simulink model "heli_q8_Part4_AI_Help"  (R2026a)
settings: Solver=ode1  StopTime=100  FixedStep=0.002  EnableMultiTasking=on
PostLoadFcn:
  | qc_set_target_type(getConfigSet(bdroot, 'QUARC Default Target Configuration'));
values from neighbouring files (symbols this model uses):
  A_d = sysd.A    [init_heli_3_10_Part4.m]    (also in init_heli_3_10_Part4_Improved.m = sysb.A; init_heli_3_10_Part4_Working.m)
  B_d = sysd.B    [init_heli_3_10_Part4.m]    (also in init_heli_3_10_Part4_Improved.m = sysb.B; init_heli_3_10_Part4_Working.m)
  C_d = sysd.C    [init_heli_3_10_Part4.m]    (also in init_heli_3_10_Part4_Improved.m = sysb.C; init_heli_3_10_Part4_Working.m)
  F = [K(1,1) K(1,3) ... (first row only)    [init_heli_3_10_Part4.m]    (also in init_heli_3_10_Part4_Improved.m; init_heli_3_10_Part4_Working.m)
  Joystick_gain_x = 1    [init_heli_3_10_Part4.m]    (also in init_heli_3_10_Part4_Improved.m; init_heli_3_10_Part4_Working.m)
  Joystick_gain_y = -1    [init_heli_3_10_Part4.m]    (also in init_heli_3_10_Part4_Improved.m; init_heli_3_10_Part4_Working.m)
  K = lqr(A_lqr,B_lqr,Q_lqr,R_lqr)    [init_heli_3_10_Part4.m]    (also in init_heli_3_10_Part4_Improved.m; init_heli_3_10_Part4_Working.m)
  K_pd = lambda_1*lambda_2/K_1    (= 7.56880733945)    [init_heli_3_10_Part4.m]    (also in init_heli_3_10_Part4_Improved.m; init_heli_3_10_Part4_Working.m)
  K_pp = - (lambda_1 + lambda_2)/K_1    (= 7.56880733945)    [init_heli_3_10_Part4.m]    (also in init_heli_3_10_Part4_Improved.m; init_heli_3_10_Part4_Working.m)
  P_0 = zeros(12)    [init_heli_3_10_Part4.m]    (also in init_heli_3_10_Part4_Improved.m = zeros(9); init_heli_3_10_Part4_Working.m)
  Q_d = Ad * Mx(1:n, n+1:end)    [init_heli_3_10_Part4.m]    (also in init_heli_3_10_Part4_Improved.m = blkdiag(Q_d6, diag([3e-12 6e-9 3e-12])); init_heli_3_10_Part4_Working.m)
  R_d2 = [R_d2 zeros(6) ... (first row only)    [init_heli_3_10_Part4.m]    (also in init_heli_3_10_Part4_Improved.m = diag(diag(R_full)); init_heli_3_10_Part4_Working.m = blkdiag(R_d2, 10^-3*R_d2))
  V_s0 = 7.5    [init_heli_3_10_Part4.m]    (also in init_heli_3_10_Part4_Improved.m; init_heli_3_10_Part4_Working.m)
  x_0 = [0;0;0;0;0;0 ... (first row only)    [init_heli_3_10_Part4.m]    (also in init_heli_3_10_Part4_Improved.m = [0; init_heli_3_10_Part4_Working.m)
undefined symbols (not defined in the file or in its folder): HIL, qc_get_step_size
libraries: quarc_library x9
settings Model: SimulationMode=external  ExtModeTrigDuration=5000  Creator=Rchan  LastModifiedBy=sandranb
settings SolverCC: PositivePriorityOrder=on
settings DataIOCC: SignalLoggingSaveFormat=ModelDataLogs
settings OptimizationCC: InitFltsAndDblsToZero=on
settings DebuggingCC: SaveWithParameterizedLinksMsg=none  UnderspecifiedInitializationDetection=Classic  MultiTaskDSMMsg=warning  MultiTaskCondExecSysMsg=none
settings HardwareCC: ProdHWDeviceType=32-bit Generic
settings RTWCC: SystemTargetFile=quarc_win64.tlc  TemplateMakefile=quarc_default_tmf  Description=QUARC Win64 Target
settings STFCustomTargetCC: SystemTargetFile=quarc_win64.tlc  TargetPreCompLibLocation=C:\PROGRA~3\QUARC\lib\2020b\win64\release  MultiwordLength=2048.0  ConcurrentExecutionCompliant=on  CPPClassGenCompliant=on  Debug=off  StopOnOverrun=off
settings GRTTargetCC: ExtMode=on  ExtModeMexFile=quarc_comm  TargetPreCompLibLocation=C:\PROGRA~3\QUARC\lib\2020b\win64\release  ParMdlRefBuildCompliant=off  CompOptLevelCompliant=off  CombineOutputUpdateFcns=off  MatFileLogging=off  GRTInterface=on

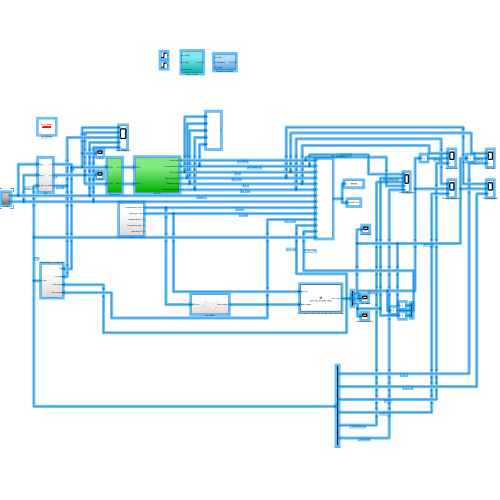
[thumbnail: Simulink's stored preview of the top-level diagram]
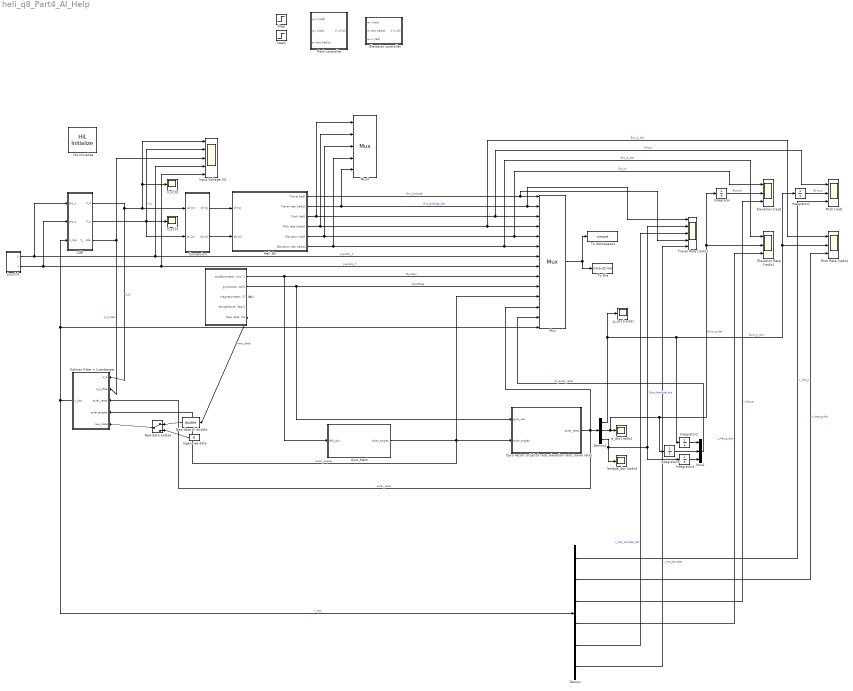
== system heli_q8_Part4_AI_Help ==
  Conversion : Subsystem
  Demux : Demux  Outputs=6
  Demux2 : Demux  Outputs=3
  Elevation Rate [rad/s] : Scope  NumInputPorts=3
      settings: ActiveDisplayYMinimum=-0.55642  ActiveDisplayYMaximum=0.56813  DataLoggingVariableName=ScopeData19
  Elevation [rad] : Scope  NumInputPorts=3
      settings: ActiveDisplayYMinimum=-0.05467  ActiveDisplayYMaximum=0.48183  DataLoggingVariableName=ScopeData18
  Elevation controller : Subsystem
  "Gyro vector to [pitch rate, elevation rate, travel rate]" : MATLAB Function  TreatAsAtomicUnit=on
  Gyro_Math : Subsystem
  HIL Initialize : quarc_library/Data Acquisition/Generic/Configuration/HIL Initialize  Priority=-99  object_name=HIL-1  board_type=q8_usb  board_number=0  board_options=update_rate=normal;decimation=1  exclusive=off  active=off  hardware_clocks=[0:2]  clock_modes=[]  initial_clock_frequencies=[]  set_clock_params_at_start=off  set_clock_params_at_switch_in=off  set_clock_frequencies_at_start=off  set_clock_frequencies_at_switch_in=off  analog_input_channels=[0:7]  analog_input_configurations=[]  analog_input_maximums=10  analog_input_minimums=-10  set_analog_input_params_at_start=on  set_analog_input_params_at_switch_in=off  analog_output_channels=[0:7]  analog_output_maximums=10  analog_output_minimums=-10  initial_analog_outputs=[0]  final_analog_outputs=[0]  watchdog_analog_outputs=0  set_analog_output_params_at_start=on  set_analog_output_params_at_switch_in=off  set_analog_outputs_at_start=on  set_analog_outputs_at_switch_in=off  set_analog_outputs_at_terminate=on  set_analog_outputs_at_switch_out=off  set_analog_outputs_on_watchdog=off  digital_input_channels=[]  digital_output_channels=[]  digital_output_configuration=[]  initial_digital_outputs=[1]  final_digital_outputs=[1]  watchdog_digital_outputs=[1]  set_digital_output_params_at_start=off  set_digital_output_params_at_switch_in=off  set_digital_outputs_at_start=on  set_digital_outputs_at_switch_in=off  set_digital_outputs_at_terminate=on  set_digital_outputs_at_switch_out=off  set_digital_outputs_on_watchdog=off  encoder_channels=[0:7]  quadrature=[4]  encoder_filter_frequency=[]  initial_encoder_counts=[0]  set_encoder_params_at_start=on  set_encoder_params_at_switch_in=off  set_encoder_counts_at_start=on  set_encoder_counts_at_switch_in=off  pwm_channels=[0:7]  pwm_modes=0  pwm_frequency=99.532799999999995e6/4095  pwm_configuration=[0]  pwm_alignment=[0]  pwm_polarity=[1]  pwm_leading_deadband=[0]  pwm_trailing_deadband=[0]  initial_pwm_outputs=[0]  final_pwm_outputs=[0]  watchdog_pwm_outputs=[0]  set_pwm_params_at_start=on  set_pwm_params_at_switch_in=off  set_pwm_outputs_at_start=on  set_pwm_outputs_at_switch_in=off  set_pwm_outputs_at_terminate=on  set_pwm_outputs_at_switch_out=off  set_pwm_outputs_on_watchdog=off  other_output_channels=[]  initial_other_outputs=[]  final_other_outputs=[]  watchdog_other_outputs=[]  set_other_outputs_at_start=off  set_other_outputs_at_switch_in=off  set_other_outputs_at_terminate=off  set_other_outputs_at_switch_out=off  set_other_outputs_on_watchdog=off
  Heli 3D : Subsystem
  IMU : Subsystem
  Input Voltage [V] : Scope  NumInputPorts=5
      settings: ActiveDisplayYMinimum=-4.40789  ActiveDisplayYMaximum=10.0852  DataLoggingVariableName=ScopeData22
  Integrator{,1..4} (5 alike) : Integrator
  Joystick : Subsystem
  Kalman Filter + Luenberger : Subsystem
  LQR : Subsystem
  Mux : Mux  Inputs=14
      settings: DisplayOption=signals
  Mux1 : Mux  Inputs=3
  Mux3 : Mux  Inputs=5
      settings: DisplayOption=signals
  Pitch Rate [rad/s] : Scope  NumInputPorts=3
      settings: ActiveDisplayYMinimum=-0.34541  ActiveDisplayYMaximum=0.52446  DataLoggingVariableName=ScopeData21
  Pitch [rad] : Scope  NumInputPorts=3
      settings: ActiveDisplayYMinimum=-0.33937  ActiveDisplayYMaximum=0.18576  DataLoggingVariableName=ScopeData20
  Pitch controller : Subsystem
  Step : Step  Time=5  FinalValue=0.5  SampleTime=0
  Step1 : Step  Time=5  FinalValue=0  SampleTime=0
  To File : ToFile  Filename=simout2.mat
  To Workspace1 : ToWorkspace  VariableName=simout  SaveFormat=Structure With Time  SampleTime=-1
  Travel Rate [rad/s] : Scope  NumInputPorts=5
      settings: ActiveDisplayYMinimum=-0.51279  ActiveDisplayYMaximum=0.73956  DataLoggingVariableName=ScopeData17
  V_d [V] : Scope
      settings: ActiveDisplayYMinimum=-0.95758  ActiveDisplayYMaximum=0.62672  DataLoggingVariableName=ScopeData13
  V_s [V] : Scope
      settings: ActiveDisplayYMinimum=-1.07949  ActiveDisplayYMaximum=9.71538  DataLoggingVariableName=ScopeData14
  e_dot [rad/s] : Scope
      settings: ActiveDisplayYMinimum=-0.55031  ActiveDisplayYMaximum=0.82946  DataLoggingVariableName=ScopeData4
  lambda_dot [rad/s] : Scope
      settings: ActiveDisplayYMinimum=-0.51279  ActiveDisplayYMaximum=0.73956  DataLoggingVariableName=ScopeData5
  p_dot [rad/s] : Scope
      settings: ActiveDisplayYMinimum=-0.32422  ActiveDisplayYMaximum=0.52211  DataLoggingVariableName=ScopeData3
  New data av/paa : ManualSwitch
  Ingen nye data : Constant  Value=0
  New data til double : DataTypeConversion  OutDataTypeStr=double  SaturateOnIntegerOverflow=off  RndMeth=Floor
  wires:
  Conversion/2(Vb [V]) -> Heli 3D/2(Vb [V])
  Conversion/1(Vf [V]) -> Heli 3D/1(Vf [V])
  Heli 3D/1(Travel [rad]) -> Travel Rate [rad/s]/4, Mux/1  "Enc_lambda"
  Heli 3D/2(Travel rate [rad/s]) -> Travel Rate [rad/s]/1, Mux/2, Mux3/5  "Enc_lambda_dot"
  Heli 3D/3(Pitch [rad]) -> Mux/3, Pitch [rad]/1, Mux3/1  "Enc_p"
  Heli 3D/4(Pitch rate [rad/s]) -> Pitch Rate [rad/s]/1, Mux/4, Mux3/2  "Enc_p_dot"
  Heli 3D/5(Elevation [rad]) -> Elevation [rad]/1, Mux/5, Mux3/3  "Enc_e"
  Heli 3D/6(Elevation rate [rad/s]) -> Elevation Rate [rad/s]/1, Mux/6, Mux3/4  "Enc_e_dot"
  Mux/1 -> To Workspace1/1, To File/1
  Joystick/1(X) -> Mux/7, Input Voltage [V]/4, LQR/1(Joy_x)  "Joystick_X"
  Joystick/2(Y) -> LQR/2(Joy_y), Mux/8, Input Voltage [V]/5  "Joystick_Y"
  IMU/1("accelerometer, m/s^2") -> Gyro_Math/1(IMU_Acc), Mux/9  "GyroAcc"
  IMU/2("gyroscope, rad/s") -> Mux/10, "Gyro vector to [pitch rate, elevation rate, travel rate]"/1(gyro_vec)  "GyroRate"
  "Gyro vector to [pitch rate, elevation rate, travel rate]"/1(euler_rates) -> Mux/12, Kalman Filter + Luenberger/3(euler_rates), Demux2/1  "euler_rates"
  Demux2/3 -> Integrator4/1, Travel Rate [rad/s]/2, lambda_dot [rad/s]/1  "Gyro_lambda_dot"
  Demux2/2 -> Integrator3/1, Elevation Rate [rad/s]/2, Integrator/1, e_dot [rad/s]/1  "Gyro_e_dot"
  Demux2/1 -> Integrator2/1, Integrator1/1, Pitch Rate [rad/s]/2, p_dot [rad/s]/1  "Gyro_p_dot"
  Gyro_Math/1(euler_angles) -> Mux/11, Kalman Filter + Luenberger/4(euler_angles), "Gyro vector to [pitch rate, elevation rate, travel rate]"/2(euler_angles)  "euler_angles"
  LQR/1(V_d) -> Conversion/1(Vd [V]), V_d [V]/1, Input Voltage [V]/1, Kalman Filter + Luenberger/1(V_d)  "V_d"
  LQR/2(V_s) -> V_s [V]/1, Conversion/2(Vs [V]), Input Voltage [V]/2  "V_s"
  Kalman Filter + Luenberger/1(x_hat) -> Mux/14, LQR/3(x_hat), Demux/1  "x_hat"
  Demux/5 -> Travel Rate [rad/s]/3  "x_hat_lambda_dot"
  Demux/3 -> Elevation [rad]/3  "x_hat_e"
  Integrator/1 -> Elevation [rad]/2  "Gyro_e"
  Demux/4 -> Elevation Rate [rad/s]/3  "x_hat_e_dot"
  Integrator1/1 -> Pitch [rad]/2  "Gyro_p"
  Demux/2 -> Pitch Rate [rad/s]/3  "x_hat_p_dot"
  Demux/1 -> Pitch [rad]/3  "x_hat_p"
  LQR/3(V_s_tilde) -> Input Voltage [V]/3, Kalman Filter + Luenberger/2(V_s_tilde)  "V_s_tilde"
  Integrator2/1 -> Mux1/1
  Integrator4/1 -> Mux1/3
  Integrator3/1 -> Mux1/2
  Mux1/1 -> Mux/13  "int_euler_rates"
  Demux/6 -> Travel Rate [rad/s]/5  "x_hat_lambda"
  IMU/5("New data, 0/1") -> New data til double/1  "new_data"
  New data til double/1 -> New data av/paa/1
  Ingen nye data/1 -> New data av/paa/2
  New data av/paa/1 -> Kalman Filter + Luenberger/5(new_data)

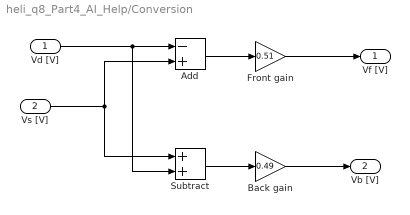
== system heli_q8_Part4_AI_Help/Conversion ==
  Vd [V] : Inport
  Vs [V] : Inport  Port=2
  Add : Sum  Inputs=-+
  Back gain : Gain  Gain=0.49
  Front gain : Gain  Gain=0.51
  Subtract : Sum
  Vf [V] : Outport
  Vb [V] : Outport  Port=2
  wires:
  Vd [V]/1 -> Subtract/2, Add/1
  Vs [V]/1 -> Subtract/1, Add/2
  Subtract/1 -> Back gain/1
  Back gain/1 -> Vb [V]/1
  Add/1 -> Front gain/1
  Front gain/1 -> Vf [V]/1

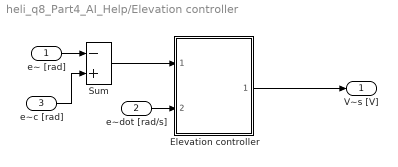
== system heli_q8_Part4_AI_Help/Elevation controller ==
  e~ [rad] : Inport
  e~dot [rad/s] : Inport  Port=2
  e~c [rad] : Inport  Port=3
  Elevation controller : Subsystem
  Sum : Sum  Inputs=-+  InputSameDT=on  SaturateOnIntegerOverflow=on  OutDataTypeStr=Inherit: Same as first input
  V~s [V] : Outport  InitialOutput=0
  wires:
  Sum/1 -> Elevation controller/1(e~ [rad])
  Elevation controller/1(V~_s [V]) -> V~s [V]/1
  e~ [rad]/1 -> Sum/1
  e~dot [rad/s]/1 -> Elevation controller/2(e~_dot [rad/s])
  e~c [rad]/1 -> Sum/2

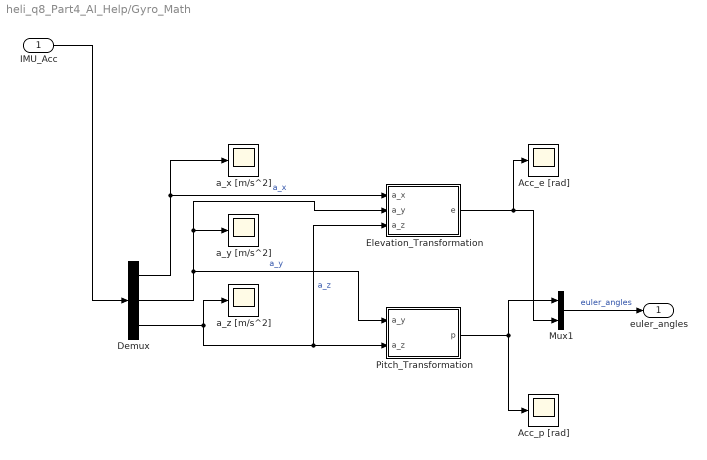
== system heli_q8_Part4_AI_Help/Gyro_Math ==
  IMU_Acc : Inport
  Acc_e [rad] : Scope
      settings: ActiveDisplayYMinimum=-0.55561  ActiveDisplayYMaximum=2.33684  DataLoggingVariableName=ScopeData2
  Acc_p [rad] : Scope
      settings: ActiveDisplayYMinimum=-0.65836  ActiveDisplayYMaximum=1.81848
  Demux : Demux  Outputs=3
  Elevation_Transformation : MATLAB Function  TreatAsAtomicUnit=on
  Mux1 : Mux  Inputs=2
  Pitch_Transformation : MATLAB Function  TreatAsAtomicUnit=on
  a_x [m/s^2] : Scope
      settings: ActiveDisplayYMinimum=-10.05504  ActiveDisplayYMaximum=6.79576
  a_y [m/s^2] : Scope
      settings: ActiveDisplayYMinimum=-2.46286  ActiveDisplayYMaximum=4.78296  DataLoggingVariableName=ScopeData2
  a_z [m/s^2] : Scope
      settings: ActiveDisplayYMinimum=-17.95765  ActiveDisplayYMaximum=1.99529  DataLoggingVariableName=ScopeData3
  euler_angles : Outport
  wires:
  Demux/1 -> a_x [m/s^2]/1, Elevation_Transformation/1(a_x)  "a_x"
  Demux/2 -> Elevation_Transformation/2(a_y), a_y [m/s^2]/1, Pitch_Transformation/1(a_y)  "a_y"
  Pitch_Transformation/1(p) -> Mux1/1, Acc_p [rad]/1
  Demux/3 -> a_z [m/s^2]/1, Elevation_Transformation/3(a_z), Pitch_Transformation/2(a_z)  "a_z"
  Elevation_Transformation/1(e) -> Acc_e [rad]/1, Mux1/2
  IMU_Acc/1 -> Demux/1
  Mux1/1 -> euler_angles/1  "euler_angles"

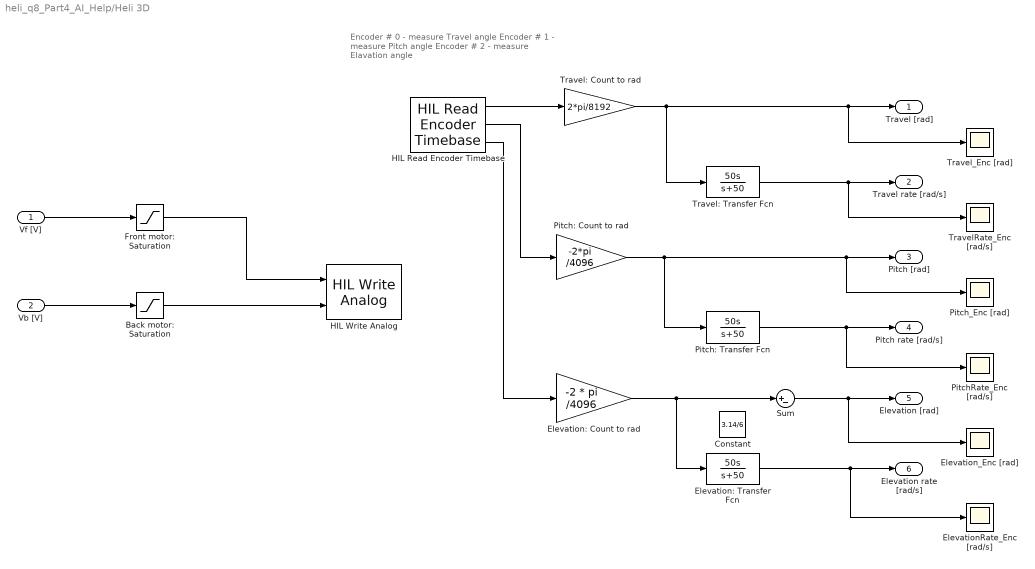
== system heli_q8_Part4_AI_Help/Heli 3D ==
  note: Encoder # 0 - measure Travel angle
      | Encoder # 1 - measure Pitch angle
      | Encoder # 2 - measure Elavation angle
  Vf [V] : Inport
  Vb [V] : Inport  Port=2
  Back motor: Saturation : Saturate  UpperLimit=5  LowerLimit=-5
  Constant : Constant  Value=3.14/6
  Elevation: Count to rad : Gain  Gain=-2 * pi /4096
  Elevation: Transfer Fcn : TransferFcn  Numerator=[50 0]  Denominator=[1 50]
  ElevationRate_Enc [rad/s] : Scope
      settings: ActiveDisplayYMinimum=-0.13148  ActiveDisplayYMaximum=0.37559  DataLoggingVariableName=ScopeData11
  Elevation_Enc [rad] : Scope
      settings: ActiveDisplayYMinimum=-0.05235  ActiveDisplayYMaximum=0.47112  DataLoggingVariableName=ScopeData10
  Front motor: Saturation : Saturate  UpperLimit=5  LowerLimit=-5
  HIL Read Encoder Timebase : quarc_library/Data Acquisition/Generic/Timebases/HIL Read Encoder Timebase  object_name=HIL-1  clock=0  channels=[0:2]  active=on  vector_output=off  data_type_mode=Inherit via back propagation  data_type=double  overflow_mode=Error on overflow  samples_in_buffer=max(ceil(1/qc_get_step_size), 1)
  HIL Write Analog : quarc_library/Data Acquisition/Generic/Immediate I//O/HIL Write Analog  object_name=HIL-1  channels=[0:1]  sample_time=-1  active=off  vector_input=off
  Pitch: Count to rad : Gain  Gain=-2*pi /4096
  Pitch: Transfer Fcn : TransferFcn  Numerator=[50 0]  Denominator=[1 50]
  PitchRate_Enc [rad/s] : Scope
      settings: ActiveDisplayYMinimum=-0.3153  ActiveDisplayYMaximum=0.25341  DataLoggingVariableName=ScopeData9
  Pitch_Enc [rad] : Scope
      settings: ActiveDisplayYMinimum=-0.33268  ActiveDisplayYMaximum=0.12559  DataLoggingVariableName=ScopeData8
  Sum : Sum  Inputs=|+-
  Travel: Count to rad : Gain  Gain=2*pi/8192
  Travel: Transfer Fcn : TransferFcn  Numerator=[50 0]  Denominator=[1 50]
  TravelRate_Enc [rad/s] : Scope
      settings: ActiveDisplayYMinimum=-0.28865  ActiveDisplayYMaximum=0.26091  DataLoggingVariableName=ScopeData7
  Travel_Enc [rad] : Scope
      settings: ActiveDisplayYMinimum=-0.31974  ActiveDisplayYMaximum=0.42328  DataLoggingVariableName=ScopeData6
  Travel [rad] : Outport
  Travel rate [rad/s] : Outport  Port=2
  Pitch [rad] : Outport  Port=3
  Pitch rate [rad/s] : Outport  Port=4
  Elevation [rad] : Outport  Port=5
  Elevation rate [rad/s] : Outport  Port=6
  wires:
  HIL Read Encoder Timebase/1 -> Travel: Count to rad/1
  HIL Read Encoder Timebase/2 -> Pitch: Count to rad/1
  HIL Read Encoder Timebase/3 -> Elevation: Count to rad/1
  Travel: Count to rad/1 -> Travel [rad]/1, Travel_Enc [rad]/1, Travel: Transfer Fcn/1
  Travel: Transfer Fcn/1 -> TravelRate_Enc [rad/s]/1, Travel rate [rad/s]/1
  Pitch: Count to rad/1 -> Pitch: Transfer Fcn/1, Pitch_Enc [rad]/1, Pitch [rad]/1
  Pitch: Transfer Fcn/1 -> PitchRate_Enc [rad/s]/1, Pitch rate [rad/s]/1
  Elevation: Count to rad/1 -> Sum/1, Elevation: Transfer Fcn/1
  Elevation: Transfer Fcn/1 -> ElevationRate_Enc [rad/s]/1, Elevation rate [rad/s]/1
  Vf [V]/1 -> Front motor: Saturation/1
  Vb [V]/1 -> Back motor: Saturation/1
  Front motor: Saturation/1 -> HIL Write Analog/1
  Back motor: Saturation/1 -> HIL Write Analog/2
  Sum/1 -> Elevation_Enc [rad]/1, Elevation [rad]/1

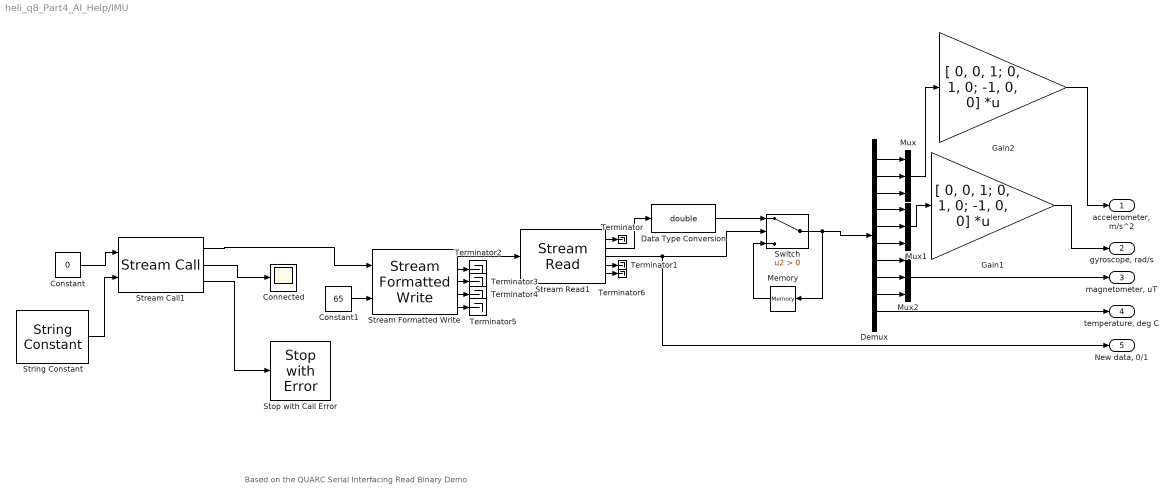
== system heli_q8_Part4_AI_Help/IMU ==
  note: Based on the QUARC Serial Interfacing Read Binary Demo
  Connected : Scope
      settings: DataLoggingVariableName=ScopeData6
  Constant : Constant  Value=0
  Constant1 : Constant  Value=65
  Data Type Conversion : DataTypeConversion  OutDataTypeStr=double  SaturateOnIntegerOverflow=off  RndMeth=Floor
  Demux : Demux  Outputs=10
  Gain1 : Gain  Gain=[ 0, 0, 1; 0, 1, 0; -1, 0, 0]  Multiplication=Matrix(K*u) (u vector)
  Gain2 : Gain  Gain=[ 0, 0, 1; 0, 1, 0; -1, 0, 0]  Multiplication=Matrix(K*u) (u vector)
  Memory : Memory  InitialCondition=[0 0 0 0 0 0 0 0 0 0]
  Mux : Mux  Inputs=3
  Mux1 : Mux  Inputs=3
  Mux2 : Mux  Inputs=3
  Stop with Call Error : quarc_library/Sinks/Error Handling/Stop with Error  message_type=Interpret input as error code  message=Error occurred
      settings: SourceProductName=QUARC Targets
  Stream Call1 : quarc_library/Communications/Intermediate/Stream Call  uri_source=External input port  uri=serial://IMU:9?baud=115200,word=8,parity=none,stop=1,flow='none'  apply_uri_to_all_configs=on  send_buffer_size=8000  receive_buffer_size=8000  byte_order=little endian (Intel - LSB first)  sample_time=qc_get_step_size  non_blocking=on  active=off
      settings: SourceProductName=QUARC Targets
  Stream Formatted Write : quarc_library/Communications/Intermediate/Stream Formatted Write  format_string=%c\n  max_code_units=80  optimization=Minimizing latency
      settings: SourceProductName=QUARC Targets
  Stream Read1 : quarc_library/Communications/Intermediate/Stream Read  data_type=single  type_expr=BusObject  num_elements=10  receive_dims=off
      settings: SourceProductName=QUARC Targets
  String Constant : quarc_library/Strings/String Constant  string_value=qc_perform_substitutions('serial://IMU:%{PORT}?baud=115200,word=8,parity=none,stop=1')  evaluate_string=on  string_type=URI  max_length=255  sample_time=inf  variable_size=off
      settings: AttributesFormatString="\"serial://IMU:6?baud=115200,word=8,parity=none,stop=1\""  SourceProductName=QUARC Targets
  Switch : Switch  Criteria=u2 > Threshold  SaturateOnIntegerOverflow=off  InputSameDT=off
  Terminator{,1..6} (7 alike) : Terminator
  "accelerometer, m/s^2" : Outport
  "gyroscope, rad/s" : Outport  Port=2
  "magnetometer, uT" : Outport  Port=3
  "temperature, deg C" : Outport  Port=4
  "New data, 0/1" : Outport  Port=5
  wires:
  Switch/1 -> Memory/1, Demux/1
  Data Type Conversion/1 -> Switch/1
  Stream Read1/3 -> "New data, 0/1"/1, Switch/2
  Stream Formatted Write/1 -> Stream Read1/1
  Constant1/1 -> Stream Formatted Write/2
  Gain1/1 -> "gyroscope, rad/s"/1
  Gain2/1 -> "accelerometer, m/s^2"/1
  Stream Read1/4 -> Terminator1/1
  Demux/10 -> "temperature, deg C"/1
  Mux1/1 -> Gain1/1
  Stream Read1/2 -> Data Type Conversion/1
  Demux/7 -> Mux2/1
  Demux/8 -> Mux2/2
  Demux/9 -> Mux2/3
  Mux2/1 -> "magnetometer, uT"/1
  Demux/6 -> Mux1/3
  Demux/5 -> Mux1/2
  Demux/4 -> Mux1/1
  Mux/1 -> Gain2/1
  Demux/3 -> Mux/3
  Demux/1 -> Mux/1
  Demux/2 -> Mux/2
  Stream Read1/1 -> Terminator/1
  Stream Call1/1 -> Stream Formatted Write/1
  Constant/1 -> Stream Call1/1
  String Constant/1 -> Stream Call1/2
  Stream Call1/2 -> Connected/1
  Stream Call1/3 -> Stop with Call Error/1
  Memory/1 -> Switch/3
  Stream Formatted Write/2 -> Terminator2/1
  Stream Formatted Write/3 -> Terminator3/1
  Stream Formatted Write/4 -> Terminator4/1
  Stream Formatted Write/5 -> Terminator5/1
  Stream Read1/5 -> Terminator6/1

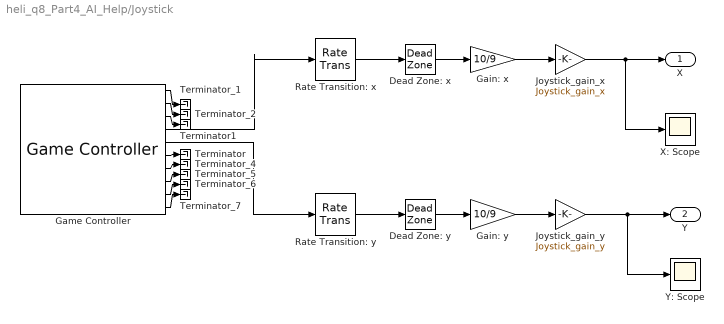
== system heli_q8_Part4_AI_Help/Joystick ==
  Dead Zone: x : DeadZone  LowerValue=-0.1  UpperValue=0.1
  Dead Zone: y : DeadZone  LowerValue=-0.1  UpperValue=0.1
  Gain: x : Gain  Gain=10/9
  Gain: y : Gain  Gain=10/9
  Game Controller : quarc_library/Devices/Peripherals/Target/Game Controller  controller=1  buffer_size=12  deadzone=[]  saturation=[]  sample_time=max(qc_get_step_size, 0.01)  auto_center=off  enabled=on
      settings: SourceProductName=QUARC Targets
  Joystick_gain_x : Gain  Gain=Joystick_gain_x
  Joystick_gain_y : Gain  Gain=Joystick_gain_y
  Rate Transition: x : RateTransition
  Rate Transition: y : RateTransition
  Terminator : Terminator
  Terminator1 : Terminator
  Terminator_{1..2,4..7} (6 alike) : Terminator
  X: Scope : Scope
      settings: ActiveDisplayYMinimum=-1  ActiveDisplayYMaximum=1  DataLoggingVariableName=ScopeData7
  Y: Scope : Scope
      settings: DataLoggingVariableName=ScopeData5
  X : Outport
  Y : Outport  Port=2
  wires:
  Rate Transition: y/1 -> Dead Zone: y/1
  Rate Transition: x/1 -> Dead Zone: x/1
  Game Controller/5 -> Rate Transition: y/1
  Game Controller/4 -> Rate Transition: x/1
  Game Controller/1 -> Terminator_1/1
  Game Controller/2 -> Terminator_2/1
  Game Controller/7 -> Terminator_4/1
  Game Controller/8 -> Terminator_5/1
  Game Controller/9 -> Terminator_6/1
  Game Controller/10 -> Terminator_7/1
  Game Controller/3 -> Terminator1/1
  Game Controller/6 -> Terminator/1
  Dead Zone: x/1 -> Gain: x/1
  Dead Zone: y/1 -> Gain: y/1
  Gain: x/1 -> Joystick_gain_x/1
  Gain: y/1 -> Joystick_gain_y/1
  Joystick_gain_x/1 -> X/1, X: Scope/1
  Joystick_gain_y/1 -> Y: Scope/1, Y/1

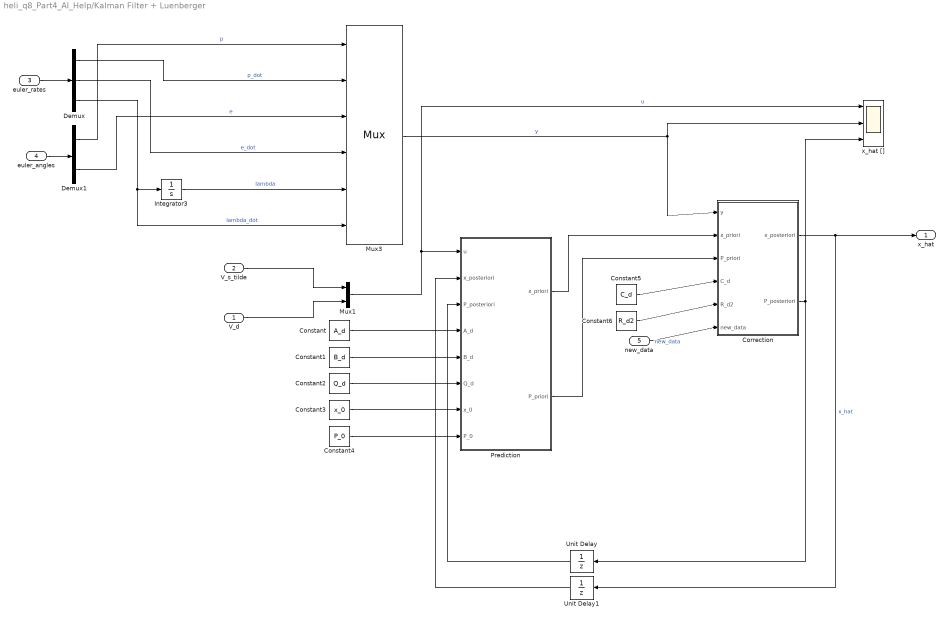
== system heli_q8_Part4_AI_Help/Kalman Filter + Luenberger ==
  V_d : Inport
  V_s_tilde : Inport  Port=2
  euler_rates : Inport  Port=3
  new_data : Inport  Port=5
  euler_angles : Inport  Port=4
  Constant : Constant  Value=A_d
  Constant1 : Constant  Value=B_d
  Constant2 : Constant  Value=Q_d
  Constant3 : Constant  Value=x_0
  Constant4 : Constant  Value=P_0
  Constant5 : Constant  Value=C_d
  Constant6 : Constant  Value=R_d2
  Correction : MATLAB Function  TreatAsAtomicUnit=on
  Demux : Demux  Outputs=3
  Demux1 : Demux  Outputs=2
  Integrator3 : Integrator
  Mux1 : Mux  Inputs=2
  Mux3 : Mux  Inputs=6
      settings: DisplayOption=signals
  Prediction : MATLAB Function  TreatAsAtomicUnit=on
  Unit Delay : UnitDelay  SampleTime=-1
  Unit Delay1 : UnitDelay  SampleTime=-1
  x_hat [] : Scope  NumInputPorts=3
      settings: ActiveDisplayYMinimum=-0.64788  ActiveDisplayYMaximum=0.72192  DataLoggingVariableName=ScopeData12
  x_hat : Outport
  wires:
  Mux3/1 -> Correction/1(y), x_hat []/2  "y"
  V_s_tilde/1 -> Mux1/1
  V_d/1 -> Mux1/2
  euler_rates/1 -> Demux/1
  Demux/1 -> Mux3/2  "p_dot"
  Demux/2 -> Mux3/4  "e_dot"
  Demux/3 -> Integrator3/1, Mux3/6  "lambda_dot"
  Integrator3/1 -> Mux3/5  "lambda"
  Mux1/1 -> x_hat []/1, Prediction/1(u)  "u"
  Prediction/1(x_priori) -> Correction/2(x_priori)
  Prediction/2(P_priori) -> Correction/3(P_priori)
  Correction/1(x_posteriori) -> Unit Delay1/1, x_hat/1  "x_hat"
  Unit Delay1/1 -> Prediction/2(x_posteriori)
  Unit Delay/1 -> Prediction/3(P_posteriori)
  Correction/2(P_posteriori) -> Unit Delay/1, x_hat []/3
  Constant/1 -> Prediction/4(A_d)
  Constant1/1 -> Prediction/5(B_d)
  Constant2/1 -> Prediction/6(Q_d)
  Constant3/1 -> Prediction/7(x_0)
  Constant4/1 -> Prediction/8(P_0)
  Constant5/1 -> Correction/4(C_d)
  Constant6/1 -> Correction/5(R_d2)
  euler_angles/1 -> Demux1/1
  Demux1/1 -> Mux3/1  "p"
  Demux1/2 -> Mux3/3  "e"
  new_data/1 -> Correction/6(new_data)  "new_data"

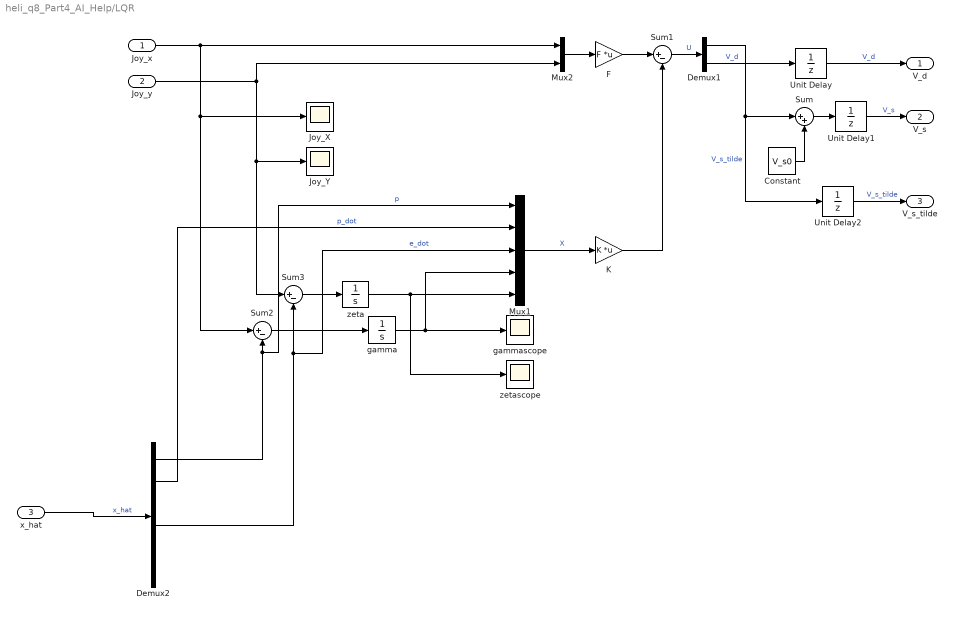
== system heli_q8_Part4_AI_Help/LQR ==
  Joy_x : Inport
  Joy_y : Inport  Port=2
  x_hat : Inport  Port=3
  Constant : Constant  Value=V_s0
  Demux1 : Demux  Outputs=2
  Demux2 : Demux  Outputs=6
  F : Gain  Gain=F  Multiplication=Matrix(K*u)
  Joy_X : Scope
      settings: ActiveDisplayYMinimum=-1  ActiveDisplayYMaximum=1
  Joy_Y : Scope
      settings: ActiveDisplayYMinimum=-1  ActiveDisplayYMaximum=1  DataLoggingVariableName=ScopeData2
  K : Gain  Gain=K  Multiplication=Matrix(K*u)
  Mux1 : Mux  Inputs=5
  Mux2 : Mux  Inputs=2
  Sum : Sum  Inputs=|++
  Sum1 : Sum  Inputs=|+-
  Sum2 : Sum  Inputs=|+-
  Sum3 : Sum  Inputs=|+-
  Unit Delay : UnitDelay  SampleTime=-1
  Unit Delay1 : UnitDelay  SampleTime=-1
  Unit Delay2 : UnitDelay  SampleTime=-1
  gamma : Integrator
  gammascope : Scope
      settings: ActiveDisplayYMinimum=-7.81453  ActiveDisplayYMaximum=1.31082  DataLoggingVariableName=ScopeData5
  zeta : Integrator
  zetascope : Scope
      settings: ActiveDisplayYMinimum=-0.42727  ActiveDisplayYMaximum=0.04825  DataLoggingVariableName=ScopeData6
  V_d : Outport
  V_s : Outport  Port=2
  V_s_tilde : Outport  Port=3
  wires:
  F/1 -> Sum1/1
  zeta/1 -> zetascope/1, Mux1/5
  gamma/1 -> Mux1/4, gammascope/1
  Sum2/1 -> gamma/1
  Mux2/1 -> F/1
  Mux1/1 -> K/1  "X"
  K/1 -> Sum1/2
  Joy_y/1 -> Mux2/2, Joy_Y/1, Sum3/1
  Sum1/1 -> Demux1/1  "U"
  Sum3/1 -> zeta/1
  Unit Delay/1 -> V_d/1  "V_d"
  Constant/1 -> Sum/2
  Demux1/1 -> Sum/1, Unit Delay2/1  "V_s_tilde"
  Sum/1 -> Unit Delay1/1
  Joy_x/1 -> Joy_X/1, Sum2/1, Mux2/1
  x_hat/1 -> Demux2/1  "x_hat"
  Demux2/4 -> Mux1/3, Sum3/2  "e_dot"
  Demux2/1 -> Mux1/1, Sum2/2  "p"
  Demux2/2 -> Mux1/2  "p_dot"
  Demux1/2 -> Unit Delay/1  "V_d"
  Unit Delay1/1 -> V_s/1  "V_s"
  Unit Delay2/1 -> V_s_tilde/1  "V_s_tilde"

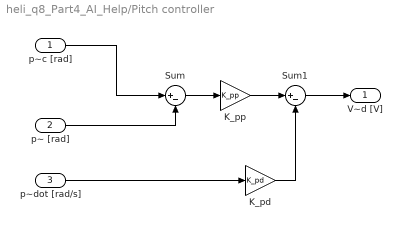
== system heli_q8_Part4_AI_Help/Pitch controller ==
  p~c [rad] : Inport
  p~ [rad] : Inport  Port=2
  p~dot [rad/s] : Inport  Port=3
  K_pd : Gain  Gain=K_pd
  K_pp : Gain  Gain=K_pp
  Sum : Sum  Inputs=|+-
  Sum1 : Sum  Inputs=|+-
  V~d [V] : Outport  InitialOutput=0
  wires:
  p~c [rad]/1 -> Sum/1
  p~ [rad]/1 -> Sum/2
  Sum/1 -> K_pp/1
  K_pp/1 -> Sum1/1
  p~dot [rad/s]/1 -> K_pd/1
  K_pd/1 -> Sum1/2
  Sum1/1 -> V~d [V]/1

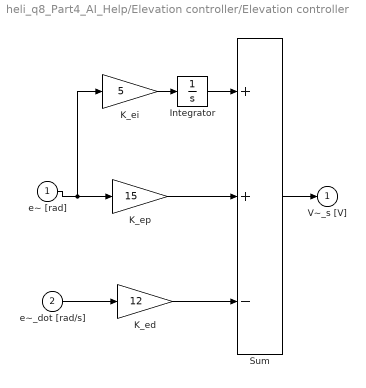
== system heli_q8_Part4_AI_Help/Elevation controller/Elevation controller ==
  e~ [rad] : Inport
  e~_dot [rad/s] : Inport  Port=2
  Integrator : Integrator  LimitOutput=on
  K_ed : Gain  Gain=12  SaturateOnIntegerOverflow=on  OutDataTypeStr=Inherit: Same as input  ParamDataTypeStr=Inherit: Same as input
  K_ei : Gain  Gain=5  SaturateOnIntegerOverflow=on  OutDataTypeStr=Inherit: Same as input  ParamDataTypeStr=Inherit: Same as input
  K_ep : Gain  Gain=15  SaturateOnIntegerOverflow=on  OutDataTypeStr=Inherit: Same as input  ParamDataTypeStr=Inherit: Same as input
  Sum : Sum  Inputs=++-  InputSameDT=on  SaturateOnIntegerOverflow=on  OutDataTypeStr=Inherit: Same as first input
  V~_s [V] : Outport  InitialOutput=0
  wires:
  K_ei/1 -> Integrator/1
  Integrator/1 -> Sum/1
  Sum/1 -> V~_s [V]/1
  e~_dot [rad/s]/1 -> K_ed/1
  K_ed/1 -> Sum/3
  K_ep/1 -> Sum/2
  e~ [rad]/1 -> K_ep/1, K_ei/1

== matlab function heli_q8_Part4_AI_Help/Gyro_Math/Elevation_Transformation ==
  data: a_x input; e output; a_y input; a_z input
function e = fcn(a_x, a_y, a_z)

N = sqrt(a_y^2+a_z^2);

if N == 0
    e = pi/2;
else
    e = atan(a_x/N);
end

== matlab function heli_q8_Part4_AI_Help/Gyro_Math/Pitch_Transformation ==
  data: a_y input; p output; a_z input
function p = fcn(a_y, a_z)

if (a_z == 0)
    p = pi/2;
else
    p = atan(a_y/a_z);
end

== matlab function heli_q8_Part4_AI_Help/Gyro vector to [pitch rate, elevation rate, travel rate] ==
  data: gyro_vec input; euler_rates output; euler_angles input
function euler_rates = gyro_vec_to_euler_rates(gyro_vec,euler_angles)
%#codegen
    phi = euler_angles(1);
    theta = euler_angles(2);
    % Hold theta unna +-pi/2 (vibrasjon ga e_acc = pi/2 og 1/cos(theta) eksploderte)
    theta = max(min(theta, 1.2), -1.2);


    T = [1, sin(phi)*tan(theta), cos(phi)*tan(theta);
         0, cos(phi),            -sin(phi);
         0, sin(phi)/cos(theta), cos(phi)/cos(theta)]; 
euler_rates = T*gyro_vec;

== matlab function heli_q8_Part4_AI_Help/Kalman Filter + Luenberger/Prediction ==
  data: u input; x_priori output; x_posteriori input; P_posteriori input; P_priori output; A_d input; B_d input; Q_d input; x_0 input; P_0 input
function [x_priori, P_priori]= fcn(u, x_posteriori, P_posteriori, A_d, B_d, Q_d, x_0, P_0)

if x_posteriori == 0
    x_posteriori = x_0;
end

if P_posteriori == 0
    P_posteriori = P_0;
end

x_priori = A_d*x_posteriori+B_d*u;
P_priori = A_d*P_posteriori*A_d' + Q_d;

== matlab function heli_q8_Part4_AI_Help/Kalman Filter + Luenberger/Correction ==
  data: y input; x_posteriori output; x_priori input; P_priori input; P_posteriori output; C_d input; R_d2 input; new_data input
function [x_posteriori, P_posteriori]= fcn(y, x_priori, P_priori, C_d, R_d2, new_data)
% Korreksjon bare naar IMU-en har levert nye data (oppgave 2.4.2).
% Uten nye data: x_hat = x_bar og P_hat = P_bar.
if new_data
    L = P_priori*C_d'/(C_d*P_priori*C_d' + R_d2);
    n = size(L,1);
    x_posteriori = x_priori + L*(y - C_d*x_priori);
    P_posteriori = (eye(n)-L*C_d)*P_priori*(eye(n)-L*C_d)' + L*R_d2*L';
else
    x_posteriori = x_priori;
    P_posteriori = P_priori;
end
